simulink model "p2_2_oscillator"  (R2025b)
settings: Solver=ode45  StartTime=0.0  StopTime=100  MaxStep=0.01  RelTol=1e-6
undefined symbols (not defined in the file or in its folder): np
settings Model: Creator=maria  LastModifiedBy=maria

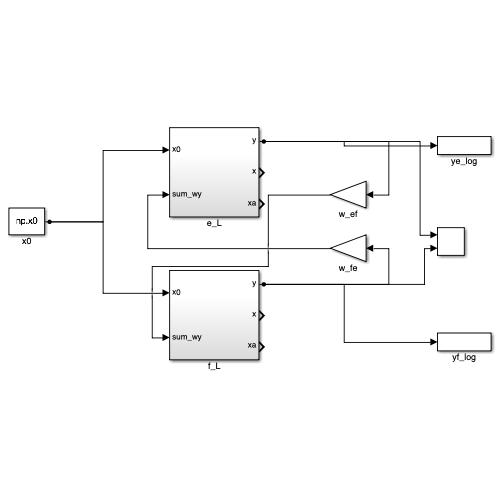
[thumbnail: Simulink's stored preview of the top-level diagram]
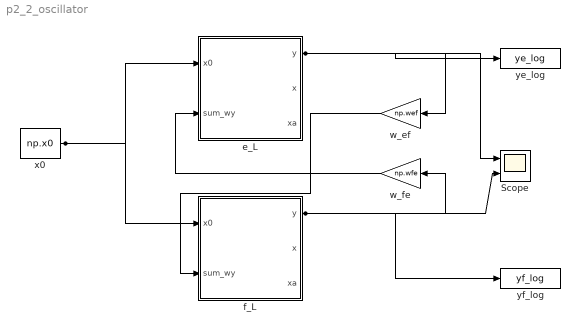
== system p2_2_oscillator ==
  Scope : Scope  NumInputPorts=2
  e_L : Subsystem
  f_L : Subsystem
  w_ef : Gain  Gain=np.wef
  w_fe : Gain  Gain=np.wfe
  x0 : Constant  Value=np.x0
  ye_log : ToWorkspace  VariableName=ye_log  SaveFormat=Timeseries  SampleTime=-1
  yf_log : ToWorkspace  VariableName=yf_log  SaveFormat=Timeseries  SampleTime=-1
  wires:
  x0/1 -> e_L/1(x0), f_L/1(x0)
  f_L/1(y) -> w_fe/1, yf_log/1, Scope/2
  w_fe/1 -> e_L/2(sum_wy)
  e_L/1(y) -> w_ef/1, ye_log/1, Scope/1
  w_ef/1 -> f_L/2(sum_wy)

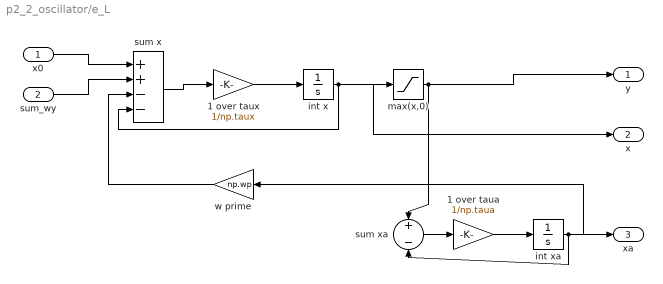
== system p2_2_oscillator/e_L ==
  x0 : Inport
  sum_wy : Inport  Port=2
  1 over taua : Gain  Gain=1/np.taua
  1 over taux : Gain  Gain=1/np.taux
  int x : Integrator  InitialCondition=1
  int xa : Integrator
  max(x,0) : Saturate  UpperLimit=inf  LowerLimit=0
  sum x : Sum  Inputs=++--
  sum xa : Sum  Inputs=+-
  w prime : Gain  Gain=np.wp
  y : Outport
  x : Outport  Port=2
  xa : Outport  Port=3
  wires:
  x0/1 -> sum x/1
  sum_wy/1 -> sum x/2
  w prime/1 -> sum x/3
  int x/1 -> sum x/4, max(x,0)/1, x/1
  sum x/1 -> 1 over taux/1
  1 over taux/1 -> int x/1
  max(x,0)/1 -> y/1, sum xa/1
  int xa/1 -> sum xa/2, xa/1, w prime/1
  sum xa/1 -> 1 over taua/1
  1 over taua/1 -> int xa/1

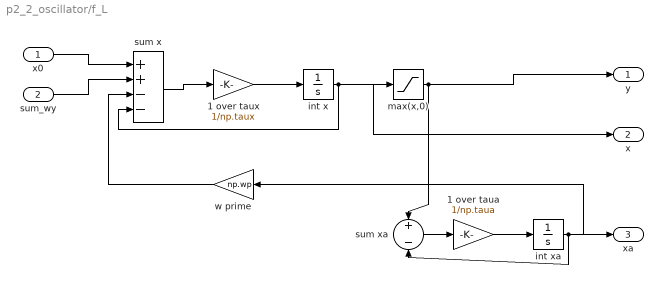
== system p2_2_oscillator/f_L ==
  x0 : Inport
  sum_wy : Inport  Port=2
  1 over taua : Gain  Gain=1/np.taua
  1 over taux : Gain  Gain=1/np.taux
  int x : Integrator
  int xa : Integrator
  max(x,0) : Saturate  UpperLimit=inf  LowerLimit=0
  sum x : Sum  Inputs=++--
  sum xa : Sum  Inputs=+-
  w prime : Gain  Gain=np.wp
  y : Outport
  x : Outport  Port=2
  xa : Outport  Port=3
  wires:
  x0/1 -> sum x/1
  sum_wy/1 -> sum x/2
  w prime/1 -> sum x/3
  int x/1 -> sum x/4, max(x,0)/1, x/1
  sum x/1 -> 1 over taux/1
  1 over taux/1 -> int x/1
  max(x,0)/1 -> y/1, sum xa/1
  int xa/1 -> sum xa/2, xa/1, w prime/1
  sum xa/1 -> 1 over taua/1
  1 over taua/1 -> int xa/1
